simulink model "My_gfm_battery_sil_12_ConvIGBT_zDomain"  (R2025b)
settings: Solver=ode23t  StartTime=0.0  StopTime=10  MaxStep=1e-4  RelTol=1e-3
PreLoadFcn:
  | close all;
  | clear all;
  | clc;
  | 
  | 
  | modelDir = fileparts(get_param(bdroot,'FileName'));
  | 
  | load_system(fullfile(modelDir,'controls_element_lib.slx'));
  | load_system(fullfile(modelDir,'test_sequence_lib.slx'));
  | 
  | Simulink.importExternalCTypes('.\circuitControls\circuitControls_A_autogen.h')
InitFcn:
  | % frequency nominals
  | F_NOM = 60;
  | W_NOM = 2 * pi * F_NOM;
  | 
  | % base values relative to inverter
  | % --------------------------------
  | VLL_INV_NOM = 480;
  | P_INV_NOM = 1e6;
  | Q_INV_NOM = 0.5e6;
  | S_INV_NOM = sqrt(P_INV_NOM^2 + Q_INV_NOM^2);
  | 
  | I_INV_BASE = S_INV_NOM/(sqrt(3)*VLL_INV_NOM);
  | Z_INV_BASE = VLL_INV_NOM^2/S_INV_NOM;
  | L_INV_BASE = Z_INV_BASE / W_NOM;
  | C_INV_BASE = 1 / (Z_INV_BASE * W_NOM);
  | 
  | % nominal ratings for power system model
  | % --------------------------------------
  | INVERTER_COUNT = 100;
  | 
  | VLV_NOM = VLL_INV_NOM;
  | VMV_NOM = 35e3;
  | VHV_NOM = 230e3;
  | S_PLANT = INVERTER_COUNT * S_INV_NOM;
  | 
  | N_GSU = VHV_NOM/VMV_NOM;
  | N_MVT = VMV_NOM/VLV_NOM;
  | 
  | I_LV_BASE = S_PLANT/(sqrt(3)*VLV_NOM);
  | I_MV_BASE = S_PLANT/(sqrt(3)*VMV_NOM);
  | I_HV_BASE = S_PLANT/(sqrt(3)*VHV_NOM);
  | 
  | Z_LV_BASE = VLV_NOM^2/S_PLANT;
  | Z_MV_BASE = VMV_NOM^2/S_PLANT;
  | Z_HV_BASE = VHV_NOM^2/S_PLANT;
  | 
  | L_LV_BASE = Z_LV_BASE / W_NOM;
  | L_MV_BASE = Z_MV_BASE / W_NOM;
  | L_HV_BASE = Z_HV_BASE / W_NOM;
  | C_LV_BASE = 1 / (Z_LV_BASE * W_NOM);
  | C_MV_BASE = 1 / (Z_MV_BASE * W_NOM);
  | C_HV_BASE = 1 / (Z_HV_BASE * W_NOM);
undefined symbols (not defined in the file): D1, D11, Delta, gcbh, j, SampleTime, sps_rtmsupport, Ts
libraries: simulink x56, spsVoltageMeasurementLib x21, spsThreePhaseSeriesRLCBranchLib x20, spsControlledCurrentSourceLib x20, spsControlledVoltageSourceLib x15, spsThreePhaseVIMeasurementLib x12, spsSeriesRLCBranchLib x11, spsGroundLib x11, test_sequence_lib x10, controls_element_lib x8, spsCurrentMeasurementLib x8, spsThreePhaseTransformerTwoWindingsLib x6
(part 2 of 9)

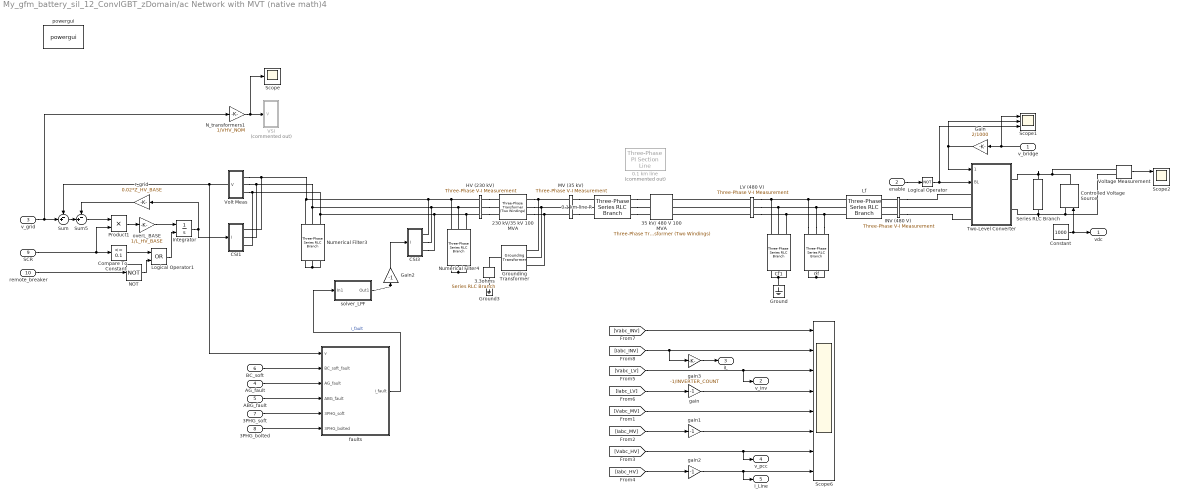
== system My_gfm_battery_sil_12_ConvIGBT_zDomain/ac Network with MVT (native math)4 ==
  v_bridge : Inport
  enable : Inport  Port=2
  v_grid : Inport  Port=3
  AG_fault : Inport  Port=4
  ABG_fault : Inport  Port=5
  BC_soft : Inport  Port=6
  3PHG_soft : Inport  Port=7
  3PHG_bolted : Inport  Port=8
  SCR : Inport  Port=9
  remote_breaker : Inport  Port=10
  0.1 km line : spsThreePhasePISectionLineLib/Three-Phase PI Section Line  Commented=on  LConnTagsString=a|b|c  RConnTagsString=A|B|C  Length=0.1  Frequency=60  Resistances=[0.1153 0.413]  Inductances=[1.05e-3 3.32e-3]  Capacitances=[11.33e-009 5.01e-009]
  0.1 km line R : spsThreePhaseSeriesRLCBranchLib/Three-Phase Series RLC Branch  LConnTagsString=A|B|C  RConnTagsString=A|B|C  BranchType=R  Resistance=0.0001  Inductance=50e-6  Capacitance=0.03*C_LV_BASE  Measurements=None
  230 kV/35 kV 100 MVA : spsThreePhaseTransformerTwoWindingsLib/Three-Phase Transformer (Two Windings)  Winding1Connection=Yg  Winding2Connection=Delta (D1)  CoreType=Three single-phase transformers  SetSaturation=off  Hysteresis=off  DataFile='basic_model'  SetInitialFlux=off  Measurements=None  UNITS=pu  NominalPower=[S_PLANT F_NOM ]  Winding1="[ VHV_NOM  0.05/50   0.05 ]"  Winding2="[ VMV_NOM  0.05/50  0.05]"  Rm=500  Lm=500  L0=0.5  Saturation="[ 0,0  ;  0.005,1.2  ;  1.0,1.4 ]"  InitialFluxes=[ 0.8 , -0.8 , 0.7 ]  BreakLoop=off  DiscreteSolver=Trapezoidal iterative  DataType=off  TransfoNumber=0
  "3.3ohms " : spsSeriesRLCBranchLib/Series RLC Branch  LConnTagsString=__new0  RConnTagsString=__new0  BranchType=R  Resistance=3.3  Inductance=[]  SetiL0=off  InitialCurrent=0  Capacitance=[]  Setx0=off  InitialVoltage=0  Measurements=None
  35 kV/ 480 V 100 MVA : spsThreePhaseTransformerTwoWindingsLib/Three-Phase Transformer (Two Windings)  Winding1Connection=Delta (D11)  Winding2Connection=Yg  CoreType=Three single-phase transformers  SetSaturation=off  Hysteresis=off  DataFile='hysteresis'  SetInitialFlux=off  Measurements=None  UNITS=pu  NominalPower="[S_PLANT  F_NOM]"  Winding1=[VMV_NOM , 0.03/50 , 0.03]  Winding2=[ VLV_NOM, 0.03/50 , 0.03]  Rm=500  Lm=500  L0=0.5  Saturation=[ 0,0 ; 0.0024,1.2 ; 1.0,1.52 ]  InitialFluxes=[ 0.8 , -0.8 , 0.7 ]  BreakLoop=off  DiscreteSolver=Trapezoidal iterative  DataType=off  TransfoNumber=0
  CSI1 : Subsystem
  CSI3 : Subsystem
  Cf : spsThreePhaseSeriesRLCBranchLib/Three-Phase Series RLC Branch  LConnTagsString=A|B|C  RConnTagsString=A|B|C  BranchType=C  Resistance=10  Inductance=1e-3  Capacitance=0.03*C_LV_BASE  Measurements=None
  Cf1 : spsThreePhaseSeriesRLCBranchLib/Three-Phase Series RLC Branch  LConnTagsString=A|B|C  RConnTagsString=A|B|C  BranchType=C  Resistance=10  Inductance=1e-3  Capacitance=0.003*C_LV_BASE  Measurements=None
  Compare To Constant : simulink/Logic and Bit Operations/Compare To Constant  relop=<=  const=0.1  OutDataTypeStr=boolean
  Constant : Constant  Value=1000
  Controlled Voltage Source : spsControlledVoltageSourceLib/Controlled Voltage Source  Initialize=off  Source_Type=AC  Amplitude=0  Phase=0  Frequency=0  Measurements=Voltage
  Gain : Gain  Gain=2/1000
  Gain2 : Gain  Gain=-1
  Ground : spsGroundLib/Ground  LConnTagsString=a
  Ground3 : spsGroundLib/Ground  LConnTagsString=a
  "Grounding Transformer " : spsGroundingTransformerLib/Grounding Transformer   UNITS=pu  NominalPower="[S_PLANT  F_NOM]"  NominalVoltage=VMV_NOM  ZeroSequenceImpedance_pu=[0.025 0.75]  MagnetizationBranch_pu=[500 500]  ZeroSequenceImpedance_SI=[0.052083 589.05]  MagnetizationBranch_SI=[1041.7 3.927e+005]  Measurements=None
  HV (230 kV) : spsThreePhaseVIMeasurementLib/Three-Phase V-I Measurement  VoltageMeasurement=phase-to-ground  SetLabelV=on  LabelV=Vabc_HV  Vpu=off  VpuLL=off  CurrentMeasurement=yes  SetLabelI=on  LabelI=Iabc_HV  Ipu=off  Pbase=S_PLANT  Vbase=VHV_NOM  OutputType=Complex  PhasorSimulation=off  PSBequivalent=0
  INV (480 V) : spsThreePhaseVIMeasurementLib/Three-Phase V-I Measurement  VoltageMeasurement=phase-to-ground  SetLabelV=on  LabelV=Vabc_INV  Vpu=off  VpuLL=off  CurrentMeasurement=yes  SetLabelI=on  LabelI=Iabc_INV  Ipu=off  Pbase=S_INV_NOM  Vbase=VLV_NOM  OutputType=Complex  PhasorSimulation=off  PSBequivalent=0
  Integrator : Integrator  ExternalReset=level
  LV (480 V) : spsThreePhaseVIMeasurementLib/Three-Phase V-I Measurement  VoltageMeasurement=phase-to-ground  SetLabelV=on  LabelV=Vabc_LV  Vpu=off  VpuLL=off  CurrentMeasurement=yes  SetLabelI=on  LabelI=Iabc_LV  Ipu=off  Pbase=S_INV_NOM  Vbase=VLV_NOM  OutputType=Complex  PhasorSimulation=off  PSBequivalent=0
  Lf : spsThreePhaseSeriesRLCBranchLib/Three-Phase Series RLC Branch  LConnTagsString=A|B|C  RConnTagsString=A|B|C  BranchType=L  Resistance=10  Inductance=0.02*L_LV_BASE  Capacitance=0.03*C_LV_BASE  Measurements=None
  Logical Operator : Logic  Operator=NOT  AllPortsSameDT=off  OutDataTypeStr=boolean
  Logical Operator1 : Logic  Operator=OR  AllPortsSameDT=off  OutDataTypeStr=boolean
  MV (35 kV) : spsThreePhaseVIMeasurementLib/Three-Phase V-I Measurement  VoltageMeasurement=phase-to-ground  SetLabelV=on  LabelV=Vabc_MV  Vpu=off  VpuLL=off  CurrentMeasurement=yes  SetLabelI=on  LabelI=Iabc_MV  Ipu=off  Pbase=S_INV_NOM  Vbase=VMV_NOM  OutputType=Complex  PhasorSimulation=off  PSBequivalent=0
  NOT : Logic  Operator=NOT  IconShape=distinctive  AllPortsSameDT=off  OutDataTypeStr=boolean
  N_transformers1 : Gain  Gain=1/VHV_NOM
  Numerical Filter3 : spsThreePhaseSeriesRLCBranchLib/Three-Phase Series RLC Branch  LConnTagsString=A|B|C  RConnTagsString=A|B|C  BranchType=R  Resistance=50*Z_HV_BASE  Inductance=50e-6  Capacitance=0.03*C_LV_BASE  Measurements=None
  Numerical Filter4 : spsThreePhaseSeriesRLCBranchLib/Three-Phase Series RLC Branch  LConnTagsString=A|B|C  RConnTagsString=A|B|C  BranchType=R  Resistance=50*Z_HV_BASE  Inductance=50e-6  Capacitance=0.03*C_LV_BASE  Measurements=None
  Product1 : Product
  Scope : Scope
      settings: ActiveDisplayYMinimum=-35721.72542  ActiveDisplayYMaximum=35721.72542
  Scope1 : Scope  NumInputPorts=3
      settings: ActiveDisplayYMinimum=-625  ActiveDisplayYMaximum=625
  Scope2 : Scope  NumInputPorts=3
      settings: ActiveDisplayYMinimum=900  ActiveDisplayYMaximum=1100  DataLoggingVariableName=ScopeData4
  Scope6 : Scope  NumInputPorts=8
      settings: ActiveDisplayYMinimum=-2828.18138  ActiveDisplayYMaximum=2137.45953  DataLoggingVariableName=ScopeData6
  Series RLC Branch : spsSeriesRLCBranchLib/Series RLC Branch  LConnTagsString=__new0  RConnTagsString=__new0  BranchType=R  Resistance=1e6  Inductance=1e-3  SetiL0=off  InitialCurrent=0  Capacitance=1e-6  Setx0=off  InitialVoltage=0  Measurements=None
  Sum : Sum  Inputs=-+|
  Sum5 : Sum  Inputs=-+|
  Two-Level Converter : Subsystem  AncestorBlock=powerlib/Power Electronics/Two-Level Converter  DialogController=POWERSYS.PowerSysDialog  LoadFcn=sps_rtmsupport('LoadFcn',gcbh);  StartFcn=sps_rtmsupport('StartFcn',gcbh);  StopFcn=sps_rtmsupport('StopFcn',gcbh);  mask(Two-Level Converter){ModelType=Average model (Uref-controlled), Ron=1e-3, Rs=1e6, Cs=inf, Vforward=[0,0], Ron_Diode=1e-3, Rs_Diode=1e3, Cs_Diode=inf, Vf_Diode=1e-3, Rs_CurrentSource=1e3}
      mask prompts: ModelType "Model type:"; Ron "Device on-state resistance (Ohms)"; Rs "Snubber resistance (Ohms)"; Cs "Snubber capacitance (F)"; Vforward "Forward voltages [Device Vf(V), Diode Vfd(V)]"; Ron_Diode "Diode on-state resistance (Ohms)"; Rs_Diode "Diode snubber resistance (Ohms)"; Cs_Diode "Diode snubber capacitance (F)"; Vf_Diode "Diode forward voltage (V)"; Rs_CurrentSource "Current source snubber resistance (Ohms)"
      mask help:
      | Implements a three-phase two-level power converter using the following modeling techniques:
      |
      | 1. Switching devices: The converter is modeled with IGBT/diode pairs controlled by firing pulses produced by a PWM generator.
      |
      | 2. Switching function: The converter is modeled by a switching function controlled by firing pulses produced by a PWM generator (0/1 signals) or by firing pulses averaged over a specified period (PWM averaging: signals between 0 and 1).
      |
      | 3. Average model (Uref-controlled): The converter is modeled using a switching-function model directly controlled by the reference voltage. A PWM generator is not required.
      |
      | Technique 1 is the most accurate, while technique 3 yields to the fastest simulation. The two techniques in 2 are well-suited for real-time simulation.
      mask init:
      | block=gcb;
      | [WantBlockChoice,Ts,BLK] = powericon('PowerConverterCback',block,Ron,Rs,Cs,Vforward,Ron_Diode,Rs_Diode,Cs_Diode,Vf_Diode,Rs_CurrentSource);
      | powericon('SetInternalModels','set',block,WantBlockChoice,3);
      settings: CopyFcn=sps_rtmsupport('CopyFcn',gcbh);  DeleteFcn=sps_rtmsupport('DeleteFcn',gcbh);  UndoDeleteFcn=sps_rtmsupport('UndoDeleteFcn',gcbh);  ModelCloseFcn=sps_rtmsupport('ModelCloseFcn',gcbh);  PreSaveFcn=sps_rtmsupport('PreSaveFcn',gcbh);  PostSaveFcn=sps_rtmsupport('PostSaveFcn',gcbh);  NameChangeFcn=sps_rtmsupport('NameChangeFcn',gcbh);  PreCopyFcn=sps_rtmsupport('PreCopyFcn',gcbh);  OpenFcn=sps_rtmsupport('OpenFcn',gcbh, [1]);  CloseFcn=sps_rtmsupport('CloseFcn',gcbh);  PreDeleteFcn=sps_rtmsupport('PreDeleteFcn',gcbh);
      mask Help: helpview(psbhelp);
      mask TypeOptions ModelType: Switching devices | Switching function | Average model (Uref-controlled)
      mask Callback ModelType: powericon('PowerConverterCback',gcb);
      mask Display:
      | x1=0.05;
      | y1=0.20;
      | %
      | plot([0.5 0.5]+x1,[0.97,0.8]-y1)
      | plot([0.5 0.32]+x1,[0.80 0.71]-y1)
      | plot([0.32 0.32]+x1,[0.80 0.52]-y1)
      | plot([0.32 0.5]+x1,[0.62 0.52]-y1)
      | plot([0.5 0.5]+x1,[0.52 0.35]-y1)
      | plot([0.45 0.5 0.43]+x1,[0.59 0.52 0.51]-y1)
      | %
      | plot([0.28 0.28]+x1,[0.74 0.58]-y1)
      | plot([0.28 0.20]+x1,[0.66 0.66]-y1)
      | %
      | plot([0.5 0.63]+x1,[0.84 0.84]-y1)
      | plot([0.63 0.63]+x1,[0.84 0.72]-y1)
      | plot([0.63 0.59]+x1,[0.72 0.65]-y1)
      | plot([0.63 0.67]+x1,[0.72 0.65]-y1)
      | plot([0.59 0.67]+x1,[0.65 0.65]-y1)
      | plot([0.63 0.63]+x1,[0.65 0.47]-y1)
      | plot([0.5 0.63]+x1,[0.47 0.47]-y1)
      | plot([0.58 0.67]+x1,[0.72 0.72]-y1)
      | %
      | color('blue')
      | text(0.3,0.1,'2-Level')
      | if ModelType==3
      |    port_label('input',1,'Uref')
      | else
      |     port_label('input',1,'g')
      | end
  VSI : Subsystem  Commented=on
  Volt Meas : Subsystem
  Voltage Measurement : spsVoltageMeasurementLib/Voltage Measurement  PhasorSimulation=off  OutputType=Complex  PSBequivalent=0
  faults : Subsystem
  gain : Gain  Gain=-1
  gain1 : Gain  Gain=-1
  gain2 : Gain  Gain=-1
  gain3 : Gain  Gain=-1/INVERTER_COUNT
  overL_BASE : Gain  Gain=1/L_HV_BASE
  powergui : spspowerguiLib/powergui  Priority=2  SimulationMode=Continuous  SampleTime=0  frequency=60  Iterations=50  frequencyindice=0  Pbase=100e6  ErrMax=1e-4  UnitsV=kV  UnitsW=MW  buscounter=0  FunctionMessages=off  echomessages=off  EnableUseOfTLC=off  CurrentSourceSwitches=off  DisableSnubberDevices=off  DisableRonSwitches=off  DisableVfSwitches=off  DisplayEquations=off  AutomaticDiscreteSolvers=off  SolverType=Tustin  Interpol=off  ExternalGateDelay=off  methode=off  Ts=0  x0status=blocks  SPID=on  SwTol=0  HookPort=off  NonlinearTolerance=1e-4  nMaxIteration=100  ContinueOnMaxIteration=off  RestoreLinks=warning  ResistiveCurrentMeasurement=off  Frange=[0:2:500]  Ylog=off  Xlog=on  ShowGrid=off  save=off  variable=ZData  structure=0  ZoomFFT=on  StartTime=0.0  cycles=1  DisplayStyle=1  fundamental=60  FreqAxis=off  MaxFrequency=1000  frequencyindicesteady=1  RmsSteady=1  display=off
  r_grid : Gain  Gain=0.02*Z_HV_BASE
  solver_LPF : Subsystem
  vdc : Outport
  v_inv : Outport  Port=2
  iL : Outport  Port=3
  v_pcc : Outport  Port=4
  i_Line : Outport  Port=5
  wires:
  AG_fault/1 -> faults/3(AG_fault)
  ABG_fault/1 -> faults/4(ABG_fault)
  BC_soft/1 -> faults/2(BC_soft_fault)
  overL_BASE/1 -> Integrator/1
  Integrator/1 -> CSI1/1(I), r_grid/1
  faults/1(i_fault) -> solver_LPF/1(In1)  "i_fault"
  3PHG_bolted/1 -> faults/6(3PHG_bolted)
  Product1/1 -> overL_BASE/1
  r_grid/1 -> Sum5/1
  Sum5/1 -> Product1/1
  Sum/1 -> Sum5/2
  3PHG_soft/1 -> faults/5(3PHG_soft)
  Volt Meas/1(V) -> faults/1(v), Sum/1
  solver_LPF/1(Out1) -> Gain2/1
  [Vabc_HV] -> v_pcc/1, Scope6/7
  [Vabc_INV] -> Scope6/1
  [Iabc_LV] -> gain/1
  [Vabc_MV] -> Scope6/5
  Constant/1 -> Controlled Voltage Source/1, vdc/1
  v_grid/1 -> N_transformers1/1, Sum/2
  [Iabc_INV] -> gain3/1, Scope6/2
  gain/1 -> Scope6/4
  [Iabc_HV] -> gain2/1
  [Iabc_MV] -> gain1/1
  gain1/1 -> Scope6/6
  gain2/1 -> i_Line/1, Scope6/8
  Gain2/1 -> CSI3/1(I)
  v_bridge/1 -> Scope1/1, Gain/1
  Gain/1 -> Two-Level Converter/1("  "), Scope1/2
  enable/1 -> Logical Operator/1
  Logical Operator/1 -> Scope1/3, Two-Level Converter/2(BL)
  N_transformers1/1 -> Scope/1, VSI/1(V)
  Voltage Measurement/1 -> Scope2/1
  [Vabc_LV] -> v_inv/1, Scope6/3
  gain3/1 -> iL/1
  remote_breaker/1 -> NOT/1
  Compare To Constant/1 -> Logical Operator1/1
  SCR/1 -> Compare To Constant/1, Product1/2
  Logical Operator1/1 -> Integrator/2
  NOT/1 -> Logical Operator1/2
  connections:
  "Grounding Transformer "/LConn1 -- 230 kV/35 kV 100 MVA/RConn1 -- MV (35 kV)/LConn1
  "Grounding Transformer "/LConn2 -- 230 kV/35 kV 100 MVA/RConn2 -- MV (35 kV)/LConn2
  "Grounding Transformer "/LConn3 -- 230 kV/35 kV 100 MVA/RConn3 -- MV (35 kV)/LConn3
  "3.3ohms "/LConn1 -- "Grounding Transformer "/RConn1
  MV (35 kV)/RConn3 -- 0.1 km line R/LConn3
  MV (35 kV)/RConn2 -- 0.1 km line R/LConn2
  "3.3ohms "/RConn1 -- Ground3/LConn1
  MV (35 kV)/RConn1 -- 0.1 km line R/LConn1
  Cf/RConn2 -- Cf/RConn1 -- Cf/RConn3
  Cf/LConn2 -- Lf/LConn2 -- LV (480 V)/RConn2 -- Cf1/LConn2
  HV (230 kV)/RConn1 -- 230 kV/35 kV 100 MVA/LConn1
  HV (230 kV)/RConn2 -- 230 kV/35 kV 100 MVA/LConn2
  HV (230 kV)/RConn3 -- 230 kV/35 kV 100 MVA/LConn3
  Cf/LConn3 -- Lf/LConn3 -- LV (480 V)/RConn3 -- Cf1/LConn3
  0.1 km line R/RConn2 -- 35 kV/ 480 V 100 MVA/LConn2
  0.1 km line R/RConn1 -- 35 kV/ 480 V 100 MVA/LConn1
  0.1 km line R/RConn3 -- 35 kV/ 480 V 100 MVA/LConn3
  Numerical Filter3/RConn2 -- Numerical Filter3/RConn1 -- Numerical Filter3/RConn3
  Numerical Filter4/RConn2 -- Numerical Filter4/RConn1 -- Numerical Filter4/RConn3
  Volt Meas/LConn2 -- Numerical Filter3/LConn2 -- Numerical Filter4/LConn2 -- HV (230 kV)/LConn2 -- CSI3/RConn2 -- CSI1/RConn2
  Numerical Filter4/LConn1 -- HV (230 kV)/LConn1 -- CSI3/RConn1 -- Numerical Filter3/LConn1 -- Volt Meas/LConn1 -- CSI1/RConn1
  Numerical Filter4/LConn3 -- HV (230 kV)/LConn3 -- CSI3/RConn3 -- Numerical Filter3/LConn3 -- Volt Meas/LConn3 -- CSI1/RConn3
  Two-Level Converter/RConn1 -- Voltage Measurement/LConn1 -- Controlled Voltage Source/RConn1 -- Series RLC Branch/LConn1
  Two-Level Converter/RConn2 -- Voltage Measurement/LConn2 -- Controlled Voltage Source/LConn1 -- Series RLC Branch/RConn1
  Cf/LConn1 -- Lf/LConn1 -- LV (480 V)/RConn1 -- Cf1/LConn1
  INV (480 V)/RConn1 -- Two-Level Converter/LConn1
  Two-Level Converter/LConn2 -- INV (480 V)/RConn2
  INV (480 V)/RConn3 -- Two-Level Converter/LConn3
  LV (480 V)/LConn1 -- 35 kV/ 480 V 100 MVA/RConn1
  LV (480 V)/LConn2 -- 35 kV/ 480 V 100 MVA/RConn2
  LV (480 V)/LConn3 -- 35 kV/ 480 V 100 MVA/RConn3
  INV (480 V)/LConn2 -- Lf/RConn2
  INV (480 V)/LConn1 -- Lf/RConn1
  INV (480 V)/LConn3 -- Lf/RConn3
  Cf1/RConn2 -- Cf1/RConn1 -- Cf1/RConn3 -- Ground/LConn1

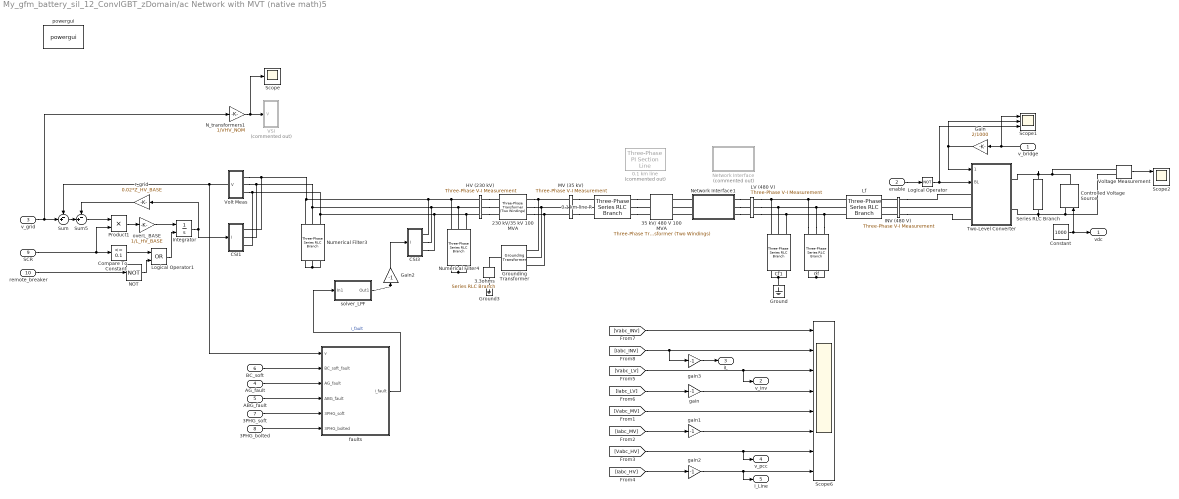
== system My_gfm_battery_sil_12_ConvIGBT_zDomain/ac Network with MVT (native math)5 ==
  v_bridge : Inport
  enable : Inport  Port=2
  v_grid : Inport  Port=3
  AG_fault : Inport  Port=4
  ABG_fault : Inport  Port=5
  BC_soft : Inport  Port=6
  3PHG_soft : Inport  Port=7
  3PHG_bolted : Inport  Port=8
  SCR : Inport  Port=9
  remote_breaker : Inport  Port=10
  0.1 km line : spsThreePhasePISectionLineLib/Three-Phase PI Section Line  Commented=on  LConnTagsString=a|b|c  RConnTagsString=A|B|C  Length=0.1  Frequency=60  Resistances=[0.1153 0.413]  Inductances=[1.05e-3 3.32e-3]  Capacitances=[11.33e-009 5.01e-009]
  0.1 km line R : spsThreePhaseSeriesRLCBranchLib/Three-Phase Series RLC Branch  LConnTagsString=A|B|C  RConnTagsString=A|B|C  BranchType=R  Resistance=0.0001  Inductance=50e-6  Capacitance=0.03*C_LV_BASE  Measurements=None
  230 kV/35 kV 100 MVA : spsThreePhaseTransformerTwoWindingsLib/Three-Phase Transformer (Two Windings)  Winding1Connection=Yg  Winding2Connection=Delta (D1)  CoreType=Three single-phase transformers  SetSaturation=off  Hysteresis=off  DataFile='basic_model'  SetInitialFlux=off  Measurements=None  UNITS=pu  NominalPower=[S_PLANT F_NOM ]  Winding1="[ VHV_NOM  0.05/50   0.05 ]"  Winding2="[ VMV_NOM  0.05/50  0.05]"  Rm=500  Lm=500  L0=0.5  Saturation="[ 0,0  ;  0.005,1.2  ;  1.0,1.4 ]"  InitialFluxes=[ 0.8 , -0.8 , 0.7 ]  BreakLoop=off  DiscreteSolver=Trapezoidal iterative  DataType=off  TransfoNumber=0
  "3.3ohms " : spsSeriesRLCBranchLib/Series RLC Branch  LConnTagsString=__new0  RConnTagsString=__new0  BranchType=R  Resistance=3.3  Inductance=[]  SetiL0=off  InitialCurrent=0  Capacitance=[]  Setx0=off  InitialVoltage=0  Measurements=None
  35 kV/ 480 V 100 MVA : spsThreePhaseTransformerTwoWindingsLib/Three-Phase Transformer (Two Windings)  Winding1Connection=Delta (D11)  Winding2Connection=Yg  CoreType=Three single-phase transformers  SetSaturation=off  Hysteresis=off  DataFile='hysteresis'  SetInitialFlux=off  Measurements=None  UNITS=pu  NominalPower="[S_PLANT  F_NOM]"  Winding1=[VMV_NOM , 0.03/50 , 0.03]  Winding2=[ VLV_NOM, 0.03/50 , 0.03]  Rm=500  Lm=500  L0=0.5  Saturation=[ 0,0 ; 0.0024,1.2 ; 1.0,1.52 ]  InitialFluxes=[ 0.8 , -0.8 , 0.7 ]  BreakLoop=off  DiscreteSolver=Trapezoidal iterative  DataType=off  TransfoNumber=0
  CSI1 : Subsystem
  CSI3 : Subsystem
  Cf : spsThreePhaseSeriesRLCBranchLib/Three-Phase Series RLC Branch  LConnTagsString=A|B|C  RConnTagsString=A|B|C  BranchType=C  Resistance=10  Inductance=1e-3  Capacitance=0.03*C_INV_BASE  Measurements=None
  Cf1 : spsThreePhaseSeriesRLCBranchLib/Three-Phase Series RLC Branch  LConnTagsString=A|B|C  RConnTagsString=A|B|C  BranchType=C  Resistance=10  Inductance=1e-3  Capacitance=0.003*C_INV_BASE  Measurements=None
  Compare To Constant : simulink/Logic and Bit Operations/Compare To Constant  relop=<=  const=0.1  OutDataTypeStr=boolean
  Constant : Constant  Value=1000
  Controlled Voltage Source : spsControlledVoltageSourceLib/Controlled Voltage Source  Initialize=off  Source_Type=AC  Amplitude=0  Phase=0  Frequency=0  Measurements=Voltage
  Gain : Gain  Gain=2/1000
  Gain2 : Gain  Gain=-1
  Ground : spsGroundLib/Ground  LConnTagsString=a
  Ground3 : spsGroundLib/Ground  LConnTagsString=a
  "Grounding Transformer " : spsGroundingTransformerLib/Grounding Transformer   UNITS=pu  NominalPower="[S_PLANT  F_NOM]"  NominalVoltage=VMV_NOM  ZeroSequenceImpedance_pu=[0.025 0.75]  MagnetizationBranch_pu=[500 500]  ZeroSequenceImpedance_SI=[0.052083 589.05]  MagnetizationBranch_SI=[1041.7 3.927e+005]  Measurements=None
  HV (230 kV) : spsThreePhaseVIMeasurementLib/Three-Phase V-I Measurement  VoltageMeasurement=phase-to-ground  SetLabelV=on  LabelV=Vabc_HV  Vpu=off  VpuLL=off  CurrentMeasurement=yes  SetLabelI=on  LabelI=Iabc_HV  Ipu=off  Pbase=S_PLANT  Vbase=VHV_NOM  OutputType=Complex  PhasorSimulation=off  PSBequivalent=0
  INV (480 V) : spsThreePhaseVIMeasurementLib/Three-Phase V-I Measurement  VoltageMeasurement=phase-to-ground  SetLabelV=on  LabelV=Vabc_INV  Vpu=off  VpuLL=off  CurrentMeasurement=yes  SetLabelI=on  LabelI=Iabc_INV  Ipu=off  Pbase=S_INV_NOM  Vbase=VLV_NOM  OutputType=Complex  PhasorSimulation=off  PSBequivalent=0
  Integrator : Integrator  ExternalReset=level
  LV (480 V) : spsThreePhaseVIMeasurementLib/Three-Phase V-I Measurement  VoltageMeasurement=phase-to-ground  SetLabelV=on  LabelV=Vabc_LV  Vpu=off  VpuLL=off  CurrentMeasurement=yes  SetLabelI=on  LabelI=Iabc_LV  Ipu=off  Pbase=S_INV_NOM  Vbase=VLV_NOM  OutputType=Complex  PhasorSimulation=off  PSBequivalent=0
  Lf : spsThreePhaseSeriesRLCBranchLib/Three-Phase Series RLC Branch  LConnTagsString=A|B|C  RConnTagsString=A|B|C  BranchType=L  Resistance=10  Inductance=0.09*L_INV_BASE  Capacitance=0.03*C_LV_BASE  Measurements=None
  Logical Operator : Logic  Operator=NOT  AllPortsSameDT=off  OutDataTypeStr=boolean
  Logical Operator1 : Logic  Operator=OR  AllPortsSameDT=off  OutDataTypeStr=boolean
  MV (35 kV) : spsThreePhaseVIMeasurementLib/Three-Phase V-I Measurement  VoltageMeasurement=phase-to-ground  SetLabelV=on  LabelV=Vabc_MV  Vpu=off  VpuLL=off  CurrentMeasurement=yes  SetLabelI=on  LabelI=Iabc_MV  Ipu=off  Pbase=S_INV_NOM  Vbase=VMV_NOM  OutputType=Complex  PhasorSimulation=off  PSBequivalent=0
  NOT : Logic  Operator=NOT  IconShape=distinctive  AllPortsSameDT=off  OutDataTypeStr=boolean
  N_transformers1 : Gain  Gain=1/VHV_NOM
  Network Interface : Subsystem  Commented=on
  Network Interface1 : Subsystem
  Numerical Filter3 : spsThreePhaseSeriesRLCBranchLib/Three-Phase Series RLC Branch  LConnTagsString=A|B|C  RConnTagsString=A|B|C  BranchType=R  Resistance=50*Z_HV_BASE  Inductance=50e-6  Capacitance=0.03*C_LV_BASE  Measurements=None
  Numerical Filter4 : spsThreePhaseSeriesRLCBranchLib/Three-Phase Series RLC Branch  LConnTagsString=A|B|C  RConnTagsString=A|B|C  BranchType=R  Resistance=50*Z_HV_BASE  Inductance=50e-6  Capacitance=0.03*C_LV_BASE  Measurements=None
  Product1 : Product
  Scope : Scope
      settings: ActiveDisplayYMinimum=-35721.72542  ActiveDisplayYMaximum=35721.72542
  Scope1 : Scope  NumInputPorts=3
      settings: ActiveDisplayYMinimum=-625  ActiveDisplayYMaximum=625
  Scope2 : Scope  NumInputPorts=3
      settings: ActiveDisplayYMinimum=900  ActiveDisplayYMaximum=1100  DataLoggingVariableName=ScopeData4
  Scope6 : Scope  NumInputPorts=8
      settings: ActiveDisplayYMinimum=-2828.18138  ActiveDisplayYMaximum=2137.45953  DataLoggingVariableName=ScopeData6
  Series RLC Branch : spsSeriesRLCBranchLib/Series RLC Branch  LConnTagsString=__new0  RConnTagsString=__new0  BranchType=R  Resistance=1e6  Inductance=1e-3  SetiL0=off  InitialCurrent=0  Capacitance=1e-6  Setx0=off  InitialVoltage=0  Measurements=None
  Sum : Sum  Inputs=-+|
  Sum5 : Sum  Inputs=-+|
  Two-Level Converter : Subsystem  AncestorBlock=powerlib/Power Electronics/Two-Level Converter  DialogController=POWERSYS.PowerSysDialog  LoadFcn=sps_rtmsupport('LoadFcn',gcbh);  StartFcn=sps_rtmsupport('StartFcn',gcbh);  StopFcn=sps_rtmsupport('StopFcn',gcbh);  mask(Two-Level Converter){ModelType=Average model (Uref-controlled), Ron=1e-3, Rs=1e6, Cs=inf, Vforward=[0,0], Ron_Diode=1e-3, Rs_Diode=1e3, Cs_Diode=inf, Vf_Diode=1e-3, Rs_CurrentSource=1e3}
      mask prompts: ModelType "Model type:"; Ron "Device on-state resistance (Ohms)"; Rs "Snubber resistance (Ohms)"; Cs "Snubber capacitance (F)"; Vforward "Forward voltages [Device Vf(V), Diode Vfd(V)]"; Ron_Diode "Diode on-state resistance (Ohms)"; Rs_Diode "Diode snubber resistance (Ohms)"; Cs_Diode "Diode snubber capacitance (F)"; Vf_Diode "Diode forward voltage (V)"; Rs_CurrentSource "Current source snubber resistance (Ohms)"
      mask help:
      | Implements a three-phase two-level power converter using the following modeling techniques:
      |
      | 1. Switching devices: The converter is modeled with IGBT/diode pairs controlled by firing pulses produced by a PWM generator.
      |
      | 2. Switching function: The converter is modeled by a switching function controlled by firing pulses produced by a PWM generator (0/1 signals) or by firing pulses averaged over a specified period (PWM averaging: signals between 0 and 1).
      |
      | 3. Average model (Uref-controlled): The converter is modeled using a switching-function model directly controlled by the reference voltage. A PWM generator is not required.
      |
      | Technique 1 is the most accurate, while technique 3 yields to the fastest simulation. The two techniques in 2 are well-suited for real-time simulation.
      mask init: same as My_gfm_battery_sil_12_ConvIGBT_zDomain/ac Network with MVT (native math)4/Two-Level Converter
      settings: CopyFcn=sps_rtmsupport('CopyFcn',gcbh);  DeleteFcn=sps_rtmsupport('DeleteFcn',gcbh);  UndoDeleteFcn=sps_rtmsupport('UndoDeleteFcn',gcbh);  ModelCloseFcn=sps_rtmsupport('ModelCloseFcn',gcbh);  PreSaveFcn=sps_rtmsupport('PreSaveFcn',gcbh);  PostSaveFcn=sps_rtmsupport('PostSaveFcn',gcbh);  NameChangeFcn=sps_rtmsupport('NameChangeFcn',gcbh);  PreCopyFcn=sps_rtmsupport('PreCopyFcn',gcbh);  OpenFcn=sps_rtmsupport('OpenFcn',gcbh, [1]);  CloseFcn=sps_rtmsupport('CloseFcn',gcbh);  PreDeleteFcn=sps_rtmsupport('PreDeleteFcn',gcbh);
      mask Help: helpview(psbhelp);
      mask TypeOptions ModelType: Switching devices | Switching function | Average model (Uref-controlled)
      mask Callback ModelType: powericon('PowerConverterCback',gcb);
      mask Display:
      | x1=0.05;
      | y1=0.20;
      | %
      | plot([0.5 0.5]+x1,[0.97,0.8]-y1)
      | plot([0.5 0.32]+x1,[0.80 0.71]-y1)
      | plot([0.32 0.32]+x1,[0.80 0.52]-y1)
      | plot([0.32 0.5]+x1,[0.62 0.52]-y1)
      | plot([0.5 0.5]+x1,[0.52 0.35]-y1)
      | plot([0.45 0.5 0.43]+x1,[0.59 0.52 0.51]-y1)
      | %
      | plot([0.28 0.28]+x1,[0.74 0.58]-y1)
      | plot([0.28 0.20]+x1,[0.66 0.66]-y1)
      | %
      | plot([0.5 0.63]+x1,[0.84 0.84]-y1)
      | plot([0.63 0.63]+x1,[0.84 0.72]-y1)
      | plot([0.63 0.59]+x1,[0.72 0.65]-y1)
      | plot([0.63 0.67]+x1,[0.72 0.65]-y1)
      | plot([0.59 0.67]+x1,[0.65 0.65]-y1)
      | plot([0.63 0.63]+x1,[0.65 0.47]-y1)
      | plot([0.5 0.63]+x1,[0.47 0.47]-y1)
      | plot([0.58 0.67]+x1,[0.72 0.72]-y1)
      | %
      | color('blue')
      | text(0.3,0.1,'2-Level')
      | if ModelType==3
      |    port_label('input',1,'Uref')
      | else
      |     port_label('input',1,'g')
      | end
  VSI : Subsystem  Commented=on
  Volt Meas : Subsystem
  Voltage Measurement : spsVoltageMeasurementLib/Voltage Measurement  PhasorSimulation=off  OutputType=Complex  PSBequivalent=0
  faults : Subsystem
  gain{,1..3} (4 alike) : Gain  Gain=-1
  overL_BASE : Gain  Gain=1/L_HV_BASE
  powergui : spspowerguiLib/powergui  Priority=2  SimulationMode=Continuous  SampleTime=0  frequency=60  Iterations=50  frequencyindice=0  Pbase=100e6  ErrMax=1e-4  UnitsV=kV  UnitsW=MW  buscounter=0  FunctionMessages=off  echomessages=off  EnableUseOfTLC=off  CurrentSourceSwitches=off  DisableSnubberDevices=off  DisableRonSwitches=off  DisableVfSwitches=off  DisplayEquations=off  AutomaticDiscreteSolvers=off  SolverType=Tustin  Interpol=off  ExternalGateDelay=off  methode=off  Ts=0  x0status=blocks  SPID=on  SwTol=0  HookPort=off  NonlinearTolerance=1e-4  nMaxIteration=100  ContinueOnMaxIteration=off  RestoreLinks=warning  ResistiveCurrentMeasurement=off  Frange=[0:2:500]  Ylog=off  Xlog=on  ShowGrid=off  save=off  variable=ZData  structure=0  ZoomFFT=on  StartTime=0.0  cycles=1  DisplayStyle=1  fundamental=60  FreqAxis=off  MaxFrequency=1000  frequencyindicesteady=1  RmsSteady=1  display=off
  r_grid : Gain  Gain=0.02*Z_HV_BASE
  solver_LPF : Subsystem
  vdc : Outport
  v_inv : Outport  Port=2
  iL : Outport  Port=3
  v_pcc : Outport  Port=4
  i_Line : Outport  Port=5
  wires:
  AG_fault/1 -> faults/3(AG_fault)
  ABG_fault/1 -> faults/4(ABG_fault)
  BC_soft/1 -> faults/2(BC_soft_fault)
  overL_BASE/1 -> Integrator/1
  Integrator/1 -> CSI1/1(I), r_grid/1
  faults/1(i_fault) -> solver_LPF/1(In1)  "i_fault"
  3PHG_bolted/1 -> faults/6(3PHG_bolted)
  Product1/1 -> overL_BASE/1
  r_grid/1 -> Sum5/1
  Sum5/1 -> Product1/1
  Sum/1 -> Sum5/2
  3PHG_soft/1 -> faults/5(3PHG_soft)
  Volt Meas/1(V) -> faults/1(v), Sum/1
  solver_LPF/1(Out1) -> Gain2/1
  [Vabc_HV] -> v_pcc/1, Scope6/7
  [Vabc_INV] -> Scope6/1
  [Iabc_LV] -> gain/1
  [Vabc_MV] -> Scope6/5
  Constant/1 -> Controlled Voltage Source/1, vdc/1
  v_grid/1 -> N_transformers1/1, Sum/2
  [Iabc_INV] -> gain3/1, Scope6/2
  gain/1 -> Scope6/4
  [Iabc_HV] -> gain2/1
  [Iabc_MV] -> gain1/1
  gain1/1 -> Scope6/6
  gain2/1 -> i_Line/1, Scope6/8
  Gain2/1 -> CSI3/1(I)
  v_bridge/1 -> Scope1/1, Gain/1
  Gain/1 -> Two-Level Converter/1("  "), Scope1/2
  enable/1 -> Logical Operator/1
  Logical Operator/1 -> Scope1/3, Two-Level Converter/2(BL)
  N_transformers1/1 -> Scope/1, VSI/1(V)
  Voltage Measurement/1 -> Scope2/1
  [Vabc_LV] -> v_inv/1, Scope6/3
  gain3/1 -> iL/1
  remote_breaker/1 -> NOT/1
  Compare To Constant/1 -> Logical Operator1/1
  SCR/1 -> Compare To Constant/1, Product1/2
  Logical Operator1/1 -> Integrator/2
  NOT/1 -> Logical Operator1/2
  connections:
  "Grounding Transformer "/LConn1 -- 230 kV/35 kV 100 MVA/RConn1 -- MV (35 kV)/LConn1
  "Grounding Transformer "/LConn2 -- 230 kV/35 kV 100 MVA/RConn2 -- MV (35 kV)/LConn2
  "Grounding Transformer "/LConn3 -- 230 kV/35 kV 100 MVA/RConn3 -- MV (35 kV)/LConn3
  "3.3ohms "/LConn1 -- "Grounding Transformer "/RConn1
  MV (35 kV)/RConn3 -- 0.1 km line R/LConn3
  MV (35 kV)/RConn2 -- 0.1 km line R/LConn2
  "3.3ohms "/RConn1 -- Ground3/LConn1
  MV (35 kV)/RConn1 -- 0.1 km line R/LConn1
  Cf/RConn2 -- Cf/RConn1 -- Cf/RConn3
  Cf/LConn2 -- Lf/LConn2 -- LV (480 V)/RConn2 -- Cf1/LConn2
  HV (230 kV)/RConn1 -- 230 kV/35 kV 100 MVA/LConn1
  HV (230 kV)/RConn2 -- 230 kV/35 kV 100 MVA/LConn2
  HV (230 kV)/RConn3 -- 230 kV/35 kV 100 MVA/LConn3
  Cf/LConn3 -- Lf/LConn3 -- LV (480 V)/RConn3 -- Cf1/LConn3
  0.1 km line R/RConn2 -- 35 kV/ 480 V 100 MVA/LConn2
  0.1 km line R/RConn1 -- 35 kV/ 480 V 100 MVA/LConn1
  0.1 km line R/RConn3 -- 35 kV/ 480 V 100 MVA/LConn3
  Numerical Filter3/RConn2 -- Numerical Filter3/RConn1 -- Numerical Filter3/RConn3
  Numerical Filter4/RConn2 -- Numerical Filter4/RConn1 -- Numerical Filter4/RConn3
  Volt Meas/LConn2 -- Numerical Filter3/LConn2 -- Numerical Filter4/LConn2 -- HV (230 kV)/LConn2 -- CSI3/RConn2 -- CSI1/RConn2
  Numerical Filter4/LConn1 -- HV (230 kV)/LConn1 -- CSI3/RConn1 -- Numerical Filter3/LConn1 -- Volt Meas/LConn1 -- CSI1/RConn1
  Numerical Filter4/LConn3 -- HV (230 kV)/LConn3 -- CSI3/RConn3 -- Numerical Filter3/LConn3 -- Volt Meas/LConn3 -- CSI1/RConn3
  Two-Level Converter/RConn1 -- Voltage Measurement/LConn1 -- Controlled Voltage Source/RConn1 -- Series RLC Branch/LConn1
  Two-Level Converter/RConn2 -- Voltage Measurement/LConn2 -- Controlled Voltage Source/LConn1 -- Series RLC Branch/RConn1
  Cf/LConn1 -- Lf/LConn1 -- LV (480 V)/RConn1 -- Cf1/LConn1
  INV (480 V)/RConn1 -- Two-Level Converter/LConn1
  Two-Level Converter/LConn2 -- INV (480 V)/RConn2
  INV (480 V)/RConn3 -- Two-Level Converter/LConn3
  Network Interface1/LConn1 -- 35 kV/ 480 V 100 MVA/RConn1
  Network Interface1/RConn1 -- LV (480 V)/LConn1
  Network Interface1/LConn2 -- 35 kV/ 480 V 100 MVA/RConn2
  Network Interface1/RConn2 -- LV (480 V)/LConn2
  Network Interface1/LConn3 -- 35 kV/ 480 V 100 MVA/RConn3
  Network Interface1/RConn3 -- LV (480 V)/LConn3
  INV (480 V)/LConn2 -- Lf/RConn2
  INV (480 V)/LConn1 -- Lf/RConn1
  INV (480 V)/LConn3 -- Lf/RConn3
  Cf1/RConn2 -- Cf1/RConn1 -- Cf1/RConn3 -- Ground/LConn1

== system My_gfm_battery_sil_12_ConvIGBT_zDomain/phasor_analysis3 ==
  v : Inport
  osc : Inport  Port=2
  Complex to Magnitude-Angle : ComplexToMagnitudeAngle
  Complex to Real-Imag : ComplexToRealImag
  Conj : Math  Operator=conj  SignedPower=on
  Gain : Gain  Gain=sqrt(2)
  Gain1 : Gain  Gain=1/3
  Gain2 : Gain  Gain=sqrt(3)
  Product3 : Product
  Real-Imag to Complex : RealImagToComplex
  Scope : Scope  NumInputPorts=4
      settings: ActiveDisplayYMinimum=-476.49042  ActiveDisplayYMaximum=517.81659  DataLoggingVariableName=ScopeData6
  Sum of Elements1 : Sum  Inputs=+
  Transfer Fcn : TransferFcn  Denominator=[0.01 1]
  Transfer Fcn1 : TransferFcn  Denominator=[0.01 1]
  magnitude : Outport
  phase : Outport  Port=2
  wires:
  Complex to Magnitude-Angle/2 -> phase/1
  Complex to Magnitude-Angle/1 -> magnitude/1
  Gain2/1 -> Complex to Magnitude-Angle/1
  Gain1/1 -> Complex to Real-Imag/1
  Gain/1 -> Scope/2, Product3/2
  Real-Imag to Complex/1 -> Gain2/1
  Conj/1 -> Gain/1
  osc/1 -> Conj/1
  Complex to Real-Imag/1 -> Transfer Fcn/1
  v/1 -> Scope/1, Product3/1
  Complex to Real-Imag/2 -> Transfer Fcn1/1
  Product3/1 -> Scope/3, Sum of Elements1/1
  Transfer Fcn/1 -> Real-Imag to Complex/1
  Sum of Elements1/1 -> Scope/4, Gain1/1
  Transfer Fcn1/1 -> Real-Imag to Complex/2

== system My_gfm_battery_sil_12_ConvIGBT_zDomain/AcMeter1/PLL_3ph ==
  ref : Inport
  Complex to Real-Imag : ComplexToRealImag
  Conj : Math  Operator=conj  SignedPower=on
  Constant : Constant  Value=120
  Gain1 : Gain  Gain=1.5
  Gain2 : Gain  Gain=4.5
  Gain3 : Gain  Gain=10e-3
  Integrator : Integrator  LimitOutput=on  UpperSaturationLimit=5  LowerSaturationLimit=-5
  Product : Product
  SOGI : Subsystem  AncestorBlock=controls_module_lib/dcVoltageRegulator_A/SOGI
  Saturation : Saturate  UpperLimit=5  LowerLimit=-5
  Sum : Sum  Inputs=+++
  Sum of Elements : Sum  Inputs=+
  Sum1 : Sum  Inputs=|+-
  Transfer Fcn : TransferFcn  Denominator=[0.02 1]
  f_nom : Constant  Value=60
  oscillator_3ph : Subsystem
  freq : Outport
  osc[3] : Outport  Port=2
  wires:
  Gain1/1 -> Saturation/1
  Conj/1 -> Complex to Real-Imag/1
  ref/1 -> Product/1
  Integrator/1 -> Sum/3, Gain3/1
  Sum1/1 -> Integrator/1
  Complex to Real-Imag/2 -> Product/2
  Gain2/1 -> Sum1/1
  oscillator_3ph/1(osc[3]) -> osc[3]/1, Conj/1
  Sum/1 -> oscillator_3ph/1(f), freq/1  "freq"
  Product/1 -> Sum of Elements/1
  Saturation/1 -> Sum/2
  SOGI/1(notch) -> Gain2/1, Gain1/1  "phase_error"
  Sum of Elements/1 -> Transfer Fcn/1
  Gain3/1 -> Sum1/2
  f_nom/1 -> Sum/1
  Transfer Fcn/1 -> SOGI/1(in)  "phase_error"
  Constant/1 -> SOGI/2(fnom)

== system My_gfm_battery_sil_12_ConvIGBT_zDomain/AcMeter1/RMS calculator ==
  in[3] : Inport
  Gain : Gain  Gain=20
  Integrator : Integrator
  Square : Math  Operator=square  SignedPower=on
  Square Root : Sqrt
  Sum : Sum  Inputs=|+-
  out[3] : Outport
  wires:
  in[3]/1 -> Square/1
  Square/1 -> Sum/1
  Gain/1 -> Integrator/1
  Square Root/1 -> out[3]/1  "Vph_rms"
  Sum/1 -> Gain/1
  Integrator/1 -> Square Root/1, Sum/2

== system My_gfm_battery_sil_12_ConvIGBT_zDomain/AcMeter1/phasor_analysis ==
  in : Inport
  osc : Inport  Port=2
  Conj : Math  Operator=conj  SignedPower=on
  Conj1 : Math  Operator=conj  SignedPower=on
  Demux : Demux  Outputs=3
  Gain1 : Gain  Gain=1/3
  Gain3 : Gain  Gain=1/3
  Mux : Mux  Inputs=3
  Product1 : Product
  Product3 : Product
  Scope : Scope  NumInputPorts=5
      settings: ActiveDisplayYMinimum=-442822.4921  ActiveDisplayYMaximum=651135.82326  DataLoggingVariableName=ScopeData5
  Sum of Elements1 : Sum  Inputs=+
  Sum of Elements2 : Sum  Inputs=+
  complex_LPF1 : Subsystem  mask{wLPF=50}
      mask prompts: wLPF "Bandwidth (rad/sec)"
  complex_LPF2 : test_sequence_lib/AcMeter/phasor_analysis/complex_LPF1  wLPF=50
  sqrt(2) : Gain  Gain=sqrt(2)
  sqrt(2)1 : Gain  Gain=sqrt(2)
  perPh : Outport
  pve : Outport  Port=2
  nve : Outport  Port=3
  wires:
  complex_LPF2/1 -> Sum of Elements2/1
  Product1/1 -> complex_LPF2/1
  complex_LPF1/1(1) -> Scope/4, perPh/1
  Product3/1 -> Sum of Elements1/1, Scope/3, complex_LPF1/1(In1)
  Sum of Elements1/1 -> Scope/5, Gain1/1
  in/1 -> Scope/1, Product3/1, Product1/1
  osc/1 -> Demux/1, Conj/1
  Conj/1 -> sqrt(2)/1
  sqrt(2)/1 -> Scope/2, Product3/2
  Gain1/1 -> pve/1
  Demux/1 -> Mux/1
  Demux/2 -> Mux/3
  Demux/3 -> Mux/2
  Mux/1 -> Conj1/1
  Conj1/1 -> sqrt(2)1/1
  sqrt(2)1/1 -> Product1/2
  Sum of Elements2/1 -> Gain3/1
  Gain3/1 -> nve/1

== system My_gfm_battery_sil_12_ConvIGBT_zDomain/AcMeter1/phasor_analysis1 ==
  in : Inport
  osc : Inport  Port=2
  Conj : Math  Operator=conj  SignedPower=on
  Conj1 : Math  Operator=conj  SignedPower=on
  Demux : Demux  Outputs=3
  Gain1 : Gain  Gain=1/3
  Gain3 : Gain  Gain=1/3
  Mux : Mux  Inputs=3
  Product1 : Product
  Product3 : Product
  Sum of Elements1 : Sum  Inputs=+
  Sum of Elements2 : Sum  Inputs=+
  complex_LPF1 : Subsystem  Commented=through  mask{wLPF=50}
      mask prompts: wLPF "Bandwidth (rad/sec)"
  complex_LPF2 : test_sequence_lib/AcMeter/phasor_analysis/complex_LPF1  wLPF=50
  sqrt(2) : Gain  Gain=sqrt(2)
  sqrt(2)1 : Gain  Gain=sqrt(2)
  perPh : Outport
  pve : Outport  Port=2
  nve : Outport  Port=3
  wires:
  complex_LPF2/1 -> Sum of Elements2/1
  Product1/1 -> complex_LPF2/1
  complex_LPF1/1(1) -> perPh/1, Sum of Elements1/1
  Product3/1 -> complex_LPF1/1(In1)
  Sum of Elements1/1 -> Gain1/1
  in/1 -> Product3/1, Product1/1
  osc/1 -> Demux/1, Conj/1
  Conj/1 -> sqrt(2)/1
  sqrt(2)/1 -> Product3/2
  Gain1/1 -> pve/1
  Demux/1 -> Mux/1
  Demux/2 -> Mux/3
  Demux/3 -> Mux/2
  Mux/1 -> Conj1/1
  Conj1/1 -> sqrt(2)1/1
  sqrt(2)1/1 -> Product1/2
  Sum of Elements2/1 -> Gain3/1
  Gain3/1 -> nve/1

== system My_gfm_battery_sil_12_ConvIGBT_zDomain/My Inverter Controller /CS ==
  Ref Mag : Inport
  f : Inport  Port=2
  phase : Inport  Port=3
  Complex to Real-Imag : ComplexToRealImag
  Gain : Gain  Gain=sqrt(2)
  Product : Product
  Terminator : Terminator
  oscillator_3ph : Subsystem
  Ref : Outport
  wires:
  phase/1 -> oscillator_3ph/2(phase)
  Ref Mag/1 -> Product/2
  Product/1 -> Ref/1
  Gain/1 -> Product/1
  f/1 -> oscillator_3ph/1(f)
  oscillator_3ph/1(osc[3]) -> Complex to Real-Imag/1
  Complex to Real-Imag/1 -> Gain/1
  Complex to Real-Imag/2 -> Terminator/1

== system My_gfm_battery_sil_12_ConvIGBT_zDomain/My Inverter Controller /Imp 1 ==
  i_L : Inport
  v_dc : Inport  Port=2
  v_ac : Inport  Port=3
  i_ref : Inport  Port=4
  enable : Inport  Port=5
  freq : Inport  Port=6
  Bus Creator : BusCreator  Inputs=6  OutDataTypeStr=Bus: circuitControls_IN_t  NonVirtualBus=on
      settings: InheritFromInputs=off
  Bus Selector : BusSelector  OutputSignals=v_bridge,v_bridge_lpf
  C Function : CFunction  OutputCode=circuitControls_isr(Tstep,&Out,&In);  StartCode=|  CodegenOutputCode=circuitControls_isr(Tstep,&Out,&In);  CodegenStartCode=|  SampleTime=SampleTime  SimCustomHeaderFile=.\circuitControls\circuitControls_A_autogen.h  SimCustomSourceFile=.\circuitControls\circuit_controls_A.c  CustomHeaderFile=.\circuitControls\circuitControls_A_autogen.h  CustomSourceFile=.\circuitControls\circuit_controls_A.c  wDamp=1.0*1 / (0.8 * Z_INV_BASE * .16 * C_INV_BASE)  gDamp=1.0 / (0.8 * Z_INV_BASE)  kSlowPath=0.45  wSlowPath=1200.0  kp=0.15  wVbridge=1200.0  VBridgeLower=-1.8 * VLL_INV_NOM / sqrt(3)  VBridgeUpper="1.8 * VLL_INV_NOM  / sqrt(3)"  Tstep=50e-6  SampleTime=-1
      StartCode=|
      | set_circuitControls_CONTROLLER_CFG_wDamp(wDamp);
      | set_circuitControls_CONTROLLER_CFG_gDamp(gDamp);
      | set_circuitControls_CONTROLLER_CFG_kSlowPath(kSlowPath);
      | set_circuitControls_CONTROLLER_CFG_wSlowPath(wSlowPath);
      | set_circuitControls_CONTROLLER_CFG_kP(kp);
      | set_circuitControls_CONTROLLER_CFG_wVbridge(wVbridge);
      | set_circuitControls_LIMITS_CFG_VBridgeLower(VBridgeLower);
      | set_circuitControls_LIMITS_CFG_VBridgeUpper(VBridgeUpper);
      CodegenStartCode=|
      | set_circuitControls_CONTROLLER_CFG_wDamp(wDamp);
      | set_circuitControls_CONTROLLER_CFG_gDamp(gDamp);
      | set_circuitControls_CONTROLLER_CFG_kSlowPath(kSlowPath);
      | set_circuitControls_CONTROLLER_CFG_wSlowPath(wSlowPath);
      | set_circuitControls_CONTROLLER_CFG_kP(kp);
      | set_circuitControls_CONTROLLER_CFG_wVbridge(wVbridge);
      | set_circuitControls_LIMITS_CFG_VBridgeLower(VBridgeLower);
      | set_circuitControls_LIMITS_CFG_VBridgeUpper(VBridgeUpper);
  v_bridge : Outport
  v_bridge_lpf : Outport  Port=2
  wires:
  Bus Selector/1 -> v_bridge/1  "<v_bridge>"
  C Function/1 -> Bus Selector/1
  Bus Creator/1 -> C Function/1
  i_L/1 -> Bus Creator/1  "i_L"
  v_dc/1 -> Bus Creator/2  "v_dc"
  v_ac/1 -> Bus Creator/3  "v_ac"
  enable/1 -> Bus Creator/5  "enable"
  i_ref/1 -> Bus Creator/4  "i_ref"
  freq/1 -> Bus Creator/6  "freq"
  Bus Selector/2 -> v_bridge_lpf/1  "<v_bridge_lpf>"
